simulink model "bimanual_Diedrichsen"  (Simulink 8.1)
settings: Solver=ode4  SolverMode=SingleTasking  StartTime=0.0  StopTime=inf  FixedStep=0.0005  RelTol=1e-3
StartFcn:
  |  warndlg('Dexterit-E models cannot run under simulation. Please compile your model and run it from within Dexterit-E.');set_param(bdroot,'SimulationCommand','stop')
undefined symbols (not defined in the file or in its folder): slselsubs
libraries: Video x3, General x3, KINARM_EP_loads x3, KINARM_general x2, KINARM_loads x2, xpclib x1
(part 3 of 3)

== matlab function Show_Mirror_Target/Embedded MATLAB Function ==
  settings: fimath=|
      | fimath(...
      | 'RoundMode', 'floor',...
      | 'OverflowMode', 'wrap',...
      | 'ProductMode', 'KeepLSB', 'ProductWordLength', 32,...
      | 'SumMode', 'KeepLSB', 'SumWordLength', 32,...
      | 'CastBeforeSum', false)
  data: target input double; VCODE output double; state input double; target_type input double; opacity input double; target_display input double; x_index input double; y_index input double; num_states input double; stateindices input double
function VCODE  = fcn(target, state, target_type, opacity, target_display, x_index, y_index, num_states, stateindices)

% VCODEs are length 70. All units in a VCODE should be SI, e.g. (m) and (rad). Elements in a VCODE are defined as follows:
%
% For all target types:
%  1: target type
%       1 - circle
%       2 - ellipse
%       3 - rectangle
%       4 - line
%       5 - triangle
%       11 - circle with label
%       12 - ellipse with label
%       13 - rectangle with label
%       14 - line with label
%       15 - triangle with label
%  2: target on/off status and target display (which display target will appear on)
%		0 - off
%		1 - on, appearing on both subject and operator displays
%       2 - on, appearing on subject display only
%       3 - on, appearing on operator display only
%  3: x position (m)
%  4: y position (m)
%  5: fill colour (RRGGBB) or texture index
%  6: stroke colour (RRGGBB) or texture index
%  7: stroke width
%  8: reserved for target background ID
%  9: opacity
%
% For circles:
%  10: radius (m)
%
% For ellipses:
%  10: major radius (m)
%  11: minor radius (m)
%  12: orientation of major axis (rad)
%
% For rectangles:
%  10: length (m)
%  11: height (m)
%  12: orientation (rad) (relative to x, y already shown)
%
% For lines:
%  10: endpoint x-axis coordinate relative to start point (m)
%  11: endpoint y-axis coordinate relative to start point (m)
%
% For triangles:
%  10: length (m)
%  11: height (m)
%  12: offset of peak from midpoint of length (m)
%  13: orientation (rad)
%
% For all labelled target types:
%  14: reserved
%  15-64: label characters (indexes in ISO 8859-1 character set)
%  65: label colour (0xRRGGBB), opacity is set by the vcode's opacity (9).
%  66: label height (m)
%  67: reserved
%  68: reserved
%  69: reserved
%  70: reserved

VCODE = zeros(1, 70);

% Set the target type.
VCODE(1) = target_type;

% Set the target on/off state. If the state input is 0, the target is off. Users of the VCODE should respect this
% as an indication that the rest of the VCODE will be uninitialized.
if (state <= 0) || (state > num_states)
	VCODE(2) = 0;  % target is off
	return;
else
	VCODE(2) = target_display;  % target is on; target displays as specified by block mask
end

% Set the target position.
VCODE(3) = target(x_index) * 0.01;  % x position (convert from (cm) in target table to (m))
VCODE(4) = target(y_index) * 0.01;  % y position (convert from (cm) in target table to (m))

% Set the fill colour. Fill colour currently comes from the GUI in RRRGGGBBB format.
if stateindices(state, 1) == 0
	VCODE(5) = -2^31;
elseif target(stateindices(state, 1)) < 0
    VCODE(5) = target(stateindices(state, 1));
else
	VCODE(5) = colourshift(target(stateindices(state, 1)));
end

% Set the stroke colour. Stroke colour currently comes from the GUI in RRRGGGBBB format.
if stateindices(state, 2) == 0
	VCODE(6) = -2^31;
elseif target(stateindices(state, 2)) < 0
    VCODE(6) = target(stateindices(state, 2));
else
	VCODE(6) = colourshift(target(stateindices(state, 2)));
end

% Set the stroke width. if target table index for stroke width is zero, then the stroke width is undefined
if stateindices(state, 3) == 0
	VCODE(7) = 0;                   % if stroke width column is 0, then stroke width is 0
elseif stateindices(state, 3) < 0
	VCODE(7) = 0.001;               % if stroke width column is -ve, then a 1mm default is chosen
else
	VCODE(7) = target(stateindices(state, 3)) * 0.01;  % if stroke width column is +ve, convert width from (cm) in target table to (m)
end

% Set the opacity value, clamping it to [0, 100].
if opacity <= 0
    VCODE(9) = 0.0;
elseif opacity >= 100
    VCODE(9) = 100.0;
else
    VCODE(9) = opacity;
end

% Set attributes specific to each target type.
if target_type == 1

    % Handle circle target:
	VCODE(10)=target(stateindices(state, 4)) * 0.01;  % radius (convert from (cm) in target table to (m))

elseif target_type == 2

    % Handle ellipse target:
	VCODE(10) = target(stateindices(state, 4)) * 0.01;  % major radius (convert from (cm) in target table to (m))
	VCODE(11) = target(stateindices(state, 5)) * 0.01;  % minor radius (convert from (cm) in target table to (m))

    if stateindices(state, 6) == 0
		VCODE(12) = 0;  % if orientation column is 0, set orientation to 0 rad
	else
		VCODE(12) = mod(target(stateindices(state, 6)), 360) * pi / 180.0;  % orientation (convert from (degrees) in target table to (rad))
    end

elseif target_type == 3

    % Handle rectangle target:
    VCODE(10) = target(stateindices(state, 4)) * 0.01;  % length (convert from (cm) in target table to (m))
    VCODE(11) = target(stateindices(state, 5)) * 0.01;  % height (convert from (cm) in target table to (m))

    if stateindices(state, 6) == 0
		VCODE(12) = 0;  % if orientation column is 0, set orientation to 0 rad
	else
		VCODE(12) = mod(target(stateindices(state, 6)), 360) * pi / 180.0;  % orientation (convert from (degrees) in target table to (rad))
    end
    
elseif target_type == 4

    % Handle line target:
    VCODE(10) = target(stateindices(state, 4)) * 0.01;  % line endpoint in x axis, relative to start (convert from (cm) in target table to (m))
    VCODE(11) = target(stateindices(state, 5)) * 0.01;  % line endpoint in y axis, relative to start (convert from (cm) in target table to (m))

elseif target_type == 5

    % Handle triangle target:
    VCODE(10) = target(stateindices(state, 4)) * 0.01;  % length (convert from (cm) in target table to (m))

    % If the height column is set to 0 then the triangle is automatically made equilateral, with the base length used as length
    % for all sides. If the height column is non-zero, separate values for height and peak offset are taken from the target table.
    if stateindices(state, 5) == 0
        VCODE(11) = sin(pi / 3.0) * VCODE(10);  % height for equilateral triangle
        VCODE(12) = 0;                          % peak offset for equilateral triangle
    else
        VCODE(11) = target(stateindices(state, 5)) * 0.01;  % height (convert from (cm) in target table to (m))
        VCODE(12) = target(stateindices(state, 6)) * 0.01;  % peak offset (convert from (cm) in target table to (m))
    end

    if stateindices(state, 7) == 0
        VCODE(13) = 0;  % if orientation column is 0, set orientation to 0 rad
    else
        VCODE(13) = mod(target(stateindices(state, 7)), 360) * pi / 180.0;  % orientation (convert from (degrees) in target table to (rad))
    end
end


% The colourshift function converts an "RRRGGGBBB" colour value to RRGBB (as an uint32).
function RRGGBBAA = colourshift(RRRGGGBBB)

blue = cast(mod(RRRGGGBBB, 1000), 'uint32');
green = cast(mod(RRRGGGBBB - blue, 1000000) / 1000, 'uint32');
red = cast((RRRGGGBBB - (green * 1000) - blue) / 1000000, 'uint32');

RRGGBBAA = bitshift(red, 16) + bitshift(green, 8) + blue;

== matlab function KINARM_2ndHandInMirrorTarget/Embedded MATLAB WhichHand ==
  settings: fimath=|
      | fimath(...
      | 'RoundMode', 'floor',...
      | 'OverflowMode', 'wrap',...
      | 'ProductMode', 'KeepLSB', 'ProductWordLength', 32,...
      | 'SumMode', 'KeepLSB', 'SumWordLength', 32,...
      | 'CastBeforeSum', false)
  data: use_dominant_hand input double; dominant_hand input double; hand output double
function hand = WhichHand(use_dominant_hand, dominant_hand)

if use_dominant_hand==1				%use the dominant hand
	hand=dominant_hand;		
else
	hand=3-dominant_hand;			%use the non-dominant hand. i.e. if dominant_hand=2, hand=1 and vice-versa
end
